simulink model "model_Lab2"  (R2024a)
settings: Solver=VariableStepAuto  StartTime=0.0  StopTime=5  RelTol=1e-3
values from neighbouring files (symbols this model uses):
  k1 = -1.9731    [evaluate_controller.m]
  T = 0.001    [evaluate_controller.m]
  tau = 0.02387    [evaluate_controller.m]    (also in system_ID_Lab1.m = 1 / (2 * zeta * wn))
undefined symbols (not defined in the file or in its folder): f0, f1, g0, g1, m0, m1, n0, n1
settings Model: Creator=michael  LastModifiedBy=michael

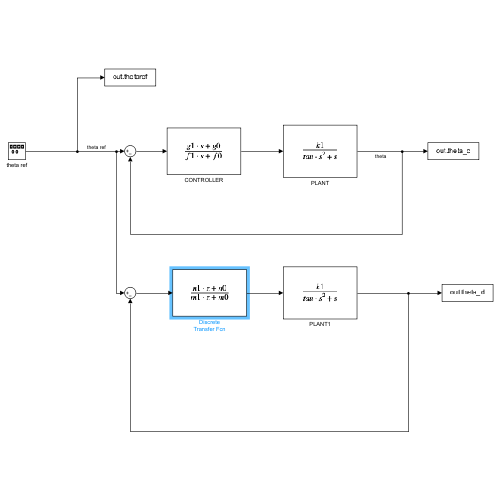
[thumbnail: Simulink's stored preview of the top-level diagram]
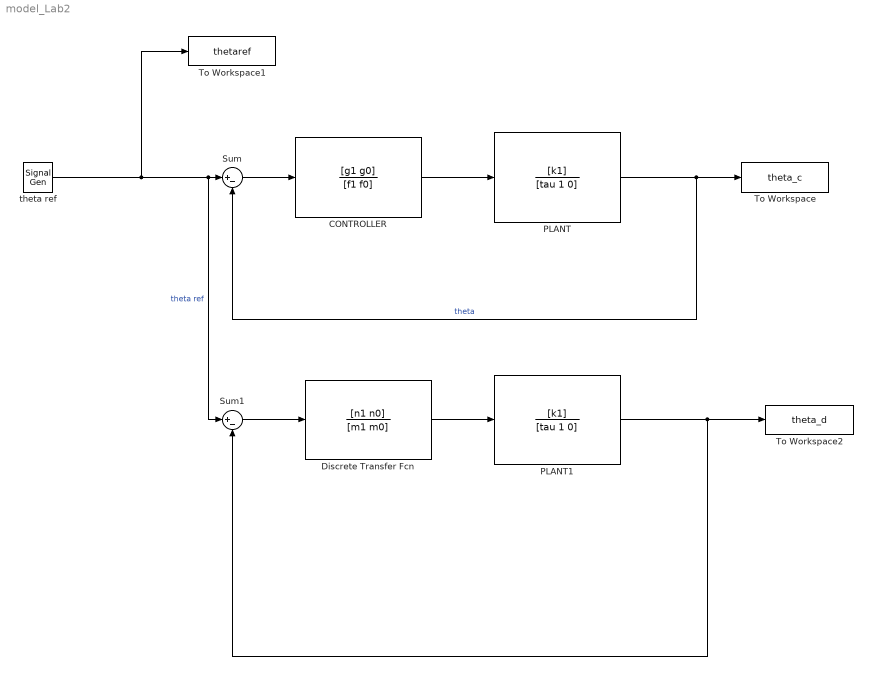
== system model_Lab2 ==
  CONTROLLER : TransferFcn  Numerator=[g1 g0]  Denominator=[f1 f0]
  Discrete Transfer Fcn : DiscreteTransferFcn  Numerator=[n1 n0]  Denominator=[m1 m0]  SampleTime=T
  PLANT : TransferFcn  Numerator=[k1]  Denominator=[tau 1 0]
  PLANT1 : TransferFcn  Numerator=[k1]  Denominator=[tau 1 0]
  Sum : Sum  Inputs=|+-
  Sum1 : Sum  Inputs=|+-
  To Workspace : ToWorkspace  VariableName=theta_c  SaveFormat=Timeseries  SampleTime=-1
  To Workspace1 : ToWorkspace  VariableName=thetaref  SaveFormat=Timeseries  SampleTime=-1
  To Workspace2 : ToWorkspace  VariableName=theta_d  SaveFormat=Timeseries  SampleTime=-1
  theta ref : SignalGenerator  WaveForm=square  Amplitude=0.7  Frequency=0.5
  wires:
  PLANT/1 -> To Workspace/1, Sum/2  "theta"
  CONTROLLER/1 -> PLANT/1
  theta ref/1 -> Sum1/1, Sum/1, To Workspace1/1  "theta ref"
  Sum/1 -> CONTROLLER/1
  Sum1/1 -> Discrete Transfer Fcn/1
  PLANT1/1 -> Sum1/2, To Workspace2/1
  Discrete Transfer Fcn/1 -> PLANT1/1
